simulink model "Copy_of_single_camera_q_dot"  (R2025b)
settings: Solver=FixedStepDiscrete  StartTime=0  StopTime=inf  FixedStep=Ts  RelTol=1e-3
InitFcn:
  | % 获取当前.slx模型所在文件夹
  | model_path = fileparts(which(gcs));
  | % 向上跳转、拼接目标函数所在文件夹（根据你的目录调整）
  | func_folder = fullfile(model_path,'..', 'config');
  | % 添加到搜索路径
  | addpath(func_folder);
  | % 执行初始化函数
  | init_single_camera_q_dot_tracking;
undefined symbols (not defined in the file or in its folder): camera_velocity_feedback_timeout_sec, controller_enable, cx, cy, data, data_SL_Info, depth_safe_max, depth_safe_min, depth_safety_gain, ekf_gate_threshold, enable_ekf_feedforward, enable_proportional, fx, fy, joint_acceleration_limit, joint_nominal_configuration, joint_position_max, joint_position_min, joint_soft_margin, joint_state_timeout_sec, joint_velocity_limit, k_ff, Kpx, Kpy, measurement_reset_timeout, nullspace_posture_gain, P0, Q_ekf, R_ekf, required_valid_frames, singularity_sigma_stop, singularity_sigma_warn, target_timeout_sec, task_velocity_filter_tau, Ts, visual_damping_max, visual_damping_min, visual_min_depth, Z_hat
libraries: ros2lib x4, robotmaniplib x2
(part 2 of 2)

== matlab function Copy_of_single_camera_q_dot/Joint State ROS2 Subscriber/Unpack ==
  data: name input; name_info input; position input; position_info input; joint_position output size=[7 1]; velocity input; velocity_info input; is_new input size=1; t input size=1; joint_count output size=1; joint_velocity output size=[7 1]; joint_age output size=1
function [joint_position,joint_count,joint_velocity,joint_age] = fcn( ...
    name,name_info,position,position_info,velocity,velocity_info,is_new,t)
%#codegen
% ROS JointState 的 name、position、velocity 使用相同索引。
% 仅当 fr3_joint1...fr3_joint7 均唯一存在且数组索引完整时才更新输出。

persistent last_q last_dq last_count last_time
if isempty(last_count)
    last_q=zeros(7,1); last_dq=zeros(7,1);
    last_count=0.0; last_time=-1.0e6;
end

if is_new
    last_q=zeros(7,1); last_dq=zeros(7,1);
    last_count=0.0; last_time=t;

    name_count=min(double(name_info.CurrentLength),double(numel(name)));
    position_count=min(double(position_info.CurrentLength),double(numel(position)));
    velocity_count=min(double(velocity_info.CurrentLength),double(numel(velocity)));

    arrays_not_truncated = ...
        double(name_info.CurrentLength)==double(name_info.ReceivedLength) && ...
        double(position_info.CurrentLength)==double(position_info.ReceivedLength) && ...
        double(velocity_info.CurrentLength)==double(velocity_info.ReceivedLength);
    message_shape_ok = arrays_not_truncated && name_count>=7.0 && ...
        position_count>=7.0 && velocity_count>=7.0;

    if message_shape_ok
        expected_names=uint8([ ...
            'fr3_joint1';'fr3_joint2';'fr3_joint3';'fr3_joint4'; ...
            'fr3_joint5';'fr3_joint6';'fr3_joint7']);
        matched=false(7,1); source_order=zeros(7,1); names_valid=true;

        for source_index=1:numel(name)
            if double(source_index)<=name_count
                character_count=min( ...
                    double(name(source_index).data_SL_Info.CurrentLength), ...
                    double(numel(name(source_index).data)));
                string_not_truncated = ...
                    double(name(source_index).data_SL_Info.CurrentLength)== ...
                    double(name(source_index).data_SL_Info.ReceivedLength);

                if string_not_truncated && character_count==10.0
                    for expected_index=1:7
                        same_name=true;
                        for character_index=1:10
                            if name(source_index).data(character_index)~= ...
                                    expected_names(expected_index,character_index)
                                same_name=false;
                            end
                        end

                        if same_name
                            if matched(expected_index)
                                names_valid=false;
                            else
                                matched(expected_index)=true;
                                source_order(expected_index)=double(source_index);
                            end
                        end
                    end
                end
            end
        end

        names_valid=names_valid && all(matched);
        indices_valid=names_valid && all(source_order>=1.0) && ...
            all(source_order<=position_count) && ...
            all(source_order<=velocity_count);

        if indices_valid
            for joint_index=1:7
                source_index=source_order(joint_index);
                last_q(joint_index)=position(source_index);
                last_dq(joint_index)=velocity(source_index);
            end

            values_valid=all(isfinite(last_q(:))) && all(isfinite(last_dq(:)));
            if values_valid
                last_count=7.0;
            else
                last_q=zeros(7,1); last_dq=zeros(7,1);
            end
        end
    end
end

joint_position=last_q; joint_count=last_count;
joint_velocity=last_dq; joint_age=max(0.0,t-last_time);
end

== matlab function Copy_of_single_camera_q_dot/Message Validation/Validate ==
  data: target_data input size=[4 1]; safe_valid output size=1; target_visible output size=1; target_count input size=1; joint_position input size=[7 1]; joint_count input size=1; joint_velocity input size=[7 1]; u output size=1; v output size=1; z output; joint_position_out output size=[7 1]; joint_velocity_out output size=[7 1]; joint_age input size=1; target_age input; joint_state_timeout_sec input; target_timeout_sec input
function [ ...
    safe_valid, ...
    target_visible, ...
    u, ...
    v, ...
    z, ...
    joint_position_out, ...
    joint_velocity_out] = fcn( ...
    target_data, ...
    target_count, ...
    joint_position, ...
    joint_count, ...
    joint_velocity, ...
    joint_age, ...
    target_age, ...
    joint_state_timeout_sec, ...
    target_timeout_sec)
%#codegen
%
% target_data：
%   (1) valid
%   (2) u，pixel
%   (3) v，pixel
%   (4) z，m

%% 1. 初始化输出

safe_valid = false;
target_visible = false;

u = 0.0;
v = 0.0;
z = 0.0;

joint_position_out = zeros(7,1);
joint_velocity_out = zeros(7,1);

%% 2. 视觉消息有效性

target_count_valid = ...
    isfinite(target_count) && ...
    target_count >= 4;

target_data_finite = ...
    all(isfinite(target_data(1:4)));

target_age_valid = ...
    isfinite(target_age) && ...
    isfinite(target_timeout_sec) && ...
    target_timeout_sec > 0.0 && ...
    target_age >= 0.0 && ...
    target_age <= target_timeout_sec;

vision_data_ok = ...
    target_count_valid && ...
    target_data_finite && ...
    target_age_valid;

%% 3. 当前是否检测到目标

target_visible = ...
    vision_data_ok && ...
    target_data(1) > 0.5;

%% 4. 关节状态有效性

joint_count_valid = ...
    isfinite(joint_count) && ...
    joint_count >= 7;

joint_pos_finite = ...
    numel(joint_position) >= 7 && ...
    all(isfinite(joint_position(1:7)));

joint_vel_finite = ...
    numel(joint_velocity) >= 7 && ...
    all(isfinite(joint_velocity(1:7)));

joint_age_valid = ...
    isfinite(joint_age) && ...
    isfinite(joint_state_timeout_sec) && ...
    joint_state_timeout_sec > 0.0 && ...
    joint_age >= 0.0 && ...
    joint_age <= joint_state_timeout_sec;

joint_ok = ...
    joint_count_valid && ...
    joint_pos_finite && ...
    joint_vel_finite && ...
    joint_age_valid;

%% 5. 输出目标数据

if target_visible
    u = target_data(2);
    v = target_data(3);
    z = target_data(4);
end

%% 6. 输出关节数据

if joint_ok
    joint_position_out = ...
        reshape(joint_position(1:7),7,1);

    joint_velocity_out = ...
        reshape(joint_velocity(1:7),7,1);
end

%% 7. 整体安全使能

safe_valid = ...
    vision_data_ok && ...
    joint_ok;

end
